simulink model "a_test"  (R2022b)
settings: Solver=VariableStepAuto  StartTime=0.0  StopTime=10.0  RelTol=1e-3
values from neighbouring files (symbols this model uses):
  L = 0.00046    [electric_current_loop.m]    (also in electric_kp_ki.m; pll.m = 10000; sl_ekf.m = c.L_LINE; sl_flux.m = L_avg - 0.5 * L_diff + L_diff * iq_obs * iq_obs / i2_obs)
undefined symbols (not defined in the file or in its folder): D_PI_I, D_PI_KB, D_PI_LOW_LIMIT, D_PI_P, D_PI_UP_LIMIT, Q_PI_I, Q_PI_KB, Q_PI_LOW_LIMIT, Q_PI_P, Q_PI_UP_LIMIT
libraries: slpidlib x6, spsPermanentMagnetSynchronousMachineLib x4, simulink x4, spsDCVoltageSourceLib x2, spsGroundLib x2, spsThreePhaseVIMeasurementLib x2, spsUniversalBridgeLib x2, spspowerguiLib x2
(part 2 of 2)

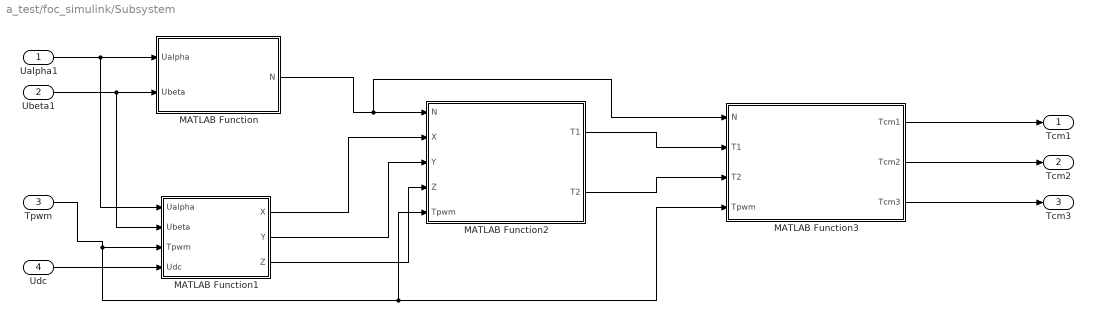
== system a_test/foc_simulink/Subsystem ==
  Ualpha1 : Inport
  Ubeta1 : Inport  Port=2
  Tpwm : Inport  Port=3
  Udc : Inport  Port=4
  MATLAB Function : MATLAB Function  TreatAsAtomicUnit=on
  MATLAB Function1 : MATLAB Function  TreatAsAtomicUnit=on
  MATLAB Function2 : MATLAB Function  TreatAsAtomicUnit=on
  MATLAB Function3 : MATLAB Function  TreatAsAtomicUnit=on
  Tcm1 : Outport
  Tcm2 : Outport  Port=2
  Tcm3 : Outport  Port=3
  wires:
  MATLAB Function3/2(Tcm2) -> Tcm2/1
  Tpwm/1 -> MATLAB Function3/4(Tpwm), MATLAB Function2/5(Tpwm), MATLAB Function1/3(Tpwm)
  MATLAB Function/1(N) -> MATLAB Function3/1(N), MATLAB Function2/1(N)
  Udc/1 -> MATLAB Function1/4(Udc)
  MATLAB Function3/3(Tcm3) -> Tcm3/1
  MATLAB Function2/1(T1) -> MATLAB Function3/2(T1)
  Ualpha1/1 -> MATLAB Function1/1(Ualpha), MATLAB Function/1(Ualpha)
  MATLAB Function2/2(T2) -> MATLAB Function3/3(T2)
  Ubeta1/1 -> MATLAB Function1/2(Ubeta), MATLAB Function/2(Ubeta)
  MATLAB Function3/1(Tcm1) -> Tcm1/1
  MATLAB Function1/1(X) -> MATLAB Function2/2(X)
  MATLAB Function1/3(Z) -> MATLAB Function2/4(Z)
  MATLAB Function1/2(Y) -> MATLAB Function2/3(Y)

== system a_test/foc_simulink/anti_park ==
  Vd : Inport
  Vq : Inport  Port=2
  theta : Inport  Port=3
  MATLAB Function : MATLAB Function  TreatAsAtomicUnit=on
  MATLAB Function1 : MATLAB Function  TreatAsAtomicUnit=on
  Valpha : Outport
  Vbeta : Outport  Port=2
  wires:
  MATLAB Function/1(Valpha) -> Valpha/1
  MATLAB Function1/1(Vbeta) -> Vbeta/1
  Vd/1 -> MATLAB Function/1(Vd), MATLAB Function1/1(Vd)
  Vq/1 -> MATLAB Function/2(Vq), MATLAB Function1/2(Vq)
  theta/1 -> MATLAB Function/3(theta), MATLAB Function1/3(theta)

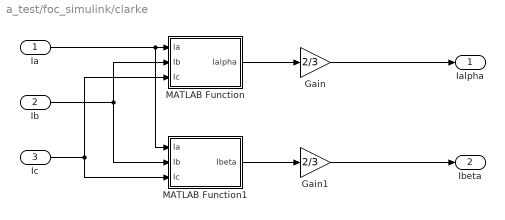
== system a_test/foc_simulink/clarke ==
  Ia : Inport
  Ib : Inport  Port=2
  Ic : Inport  Port=3
  Gain : Gain  Gain=2/3  OutDataTypeStr=single
  Gain1 : Gain  Gain=2/3  OutDataTypeStr=single
  MATLAB Function : MATLAB Function  TreatAsAtomicUnit=on
  MATLAB Function1 : MATLAB Function  TreatAsAtomicUnit=on
  Ialpha : Outport
  Ibeta : Outport  Port=2
  wires:
  Ia/1 -> MATLAB Function1/1(Ia), MATLAB Function/1(Ia)
  MATLAB Function/1(Ialpha) -> Gain/1
  Gain1/1 -> Ibeta/1
  Ib/1 -> MATLAB Function1/2(Ib), MATLAB Function/2(Ib)
  Ic/1 -> MATLAB Function/3(Ic), MATLAB Function1/3(Ic)
  MATLAB Function1/1(Ibeta) -> Gain1/1
  Gain/1 -> Ialpha/1

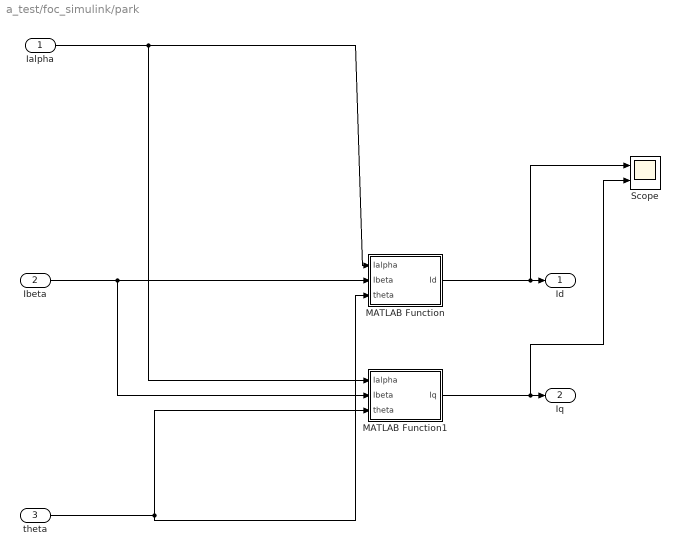
== system a_test/foc_simulink/park ==
  Ialpha : Inport
  Ibeta : Inport  Port=2
  theta : Inport  Port=3
  MATLAB Function : MATLAB Function  TreatAsAtomicUnit=on
  MATLAB Function1 : MATLAB Function  TreatAsAtomicUnit=on
  Scope : Scope  NumInputPorts=2
  Id : Outport
  Iq : Outport  Port=2
  wires:
  theta/1 -> MATLAB Function/3(theta), MATLAB Function1/3(theta)
  Ibeta/1 -> MATLAB Function/2(Ibeta), MATLAB Function1/2(Ibeta)
  MATLAB Function1/1(Iq) -> Scope/2, Iq/1
  MATLAB Function/1(Id) -> Scope/1, Id/1
  Ialpha/1 -> MATLAB Function/1(Ialpha), MATLAB Function1/1(Ialpha)

== system a_test/foc_simulink1/anti_park ==
  Vd : Inport
  Vq : Inport  Port=2
  theta : Inport  Port=3
  antipark_valpha_fun : MATLAB Function  TreatAsAtomicUnit=on
  antipark_vbeta_fun : MATLAB Function  TreatAsAtomicUnit=on
  Valpha : Outport
  Vbeta : Outport  Port=2
  wires:
  antipark_valpha_fun/1(Valpha) -> Valpha/1
  antipark_vbeta_fun/1(Vbeta) -> Vbeta/1
  Vd/1 -> antipark_valpha_fun/1(Vd), antipark_vbeta_fun/1(Vd)
  Vq/1 -> antipark_valpha_fun/2(Vq), antipark_vbeta_fun/2(Vq)
  theta/1 -> antipark_valpha_fun/3(theta), antipark_vbeta_fun/3(theta)

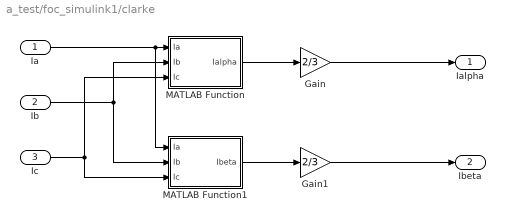
== system a_test/foc_simulink1/clarke ==
  Ia : Inport
  Ib : Inport  Port=2
  Ic : Inport  Port=3
  Gain : Gain  Gain=2/3  OutDataTypeStr=single
  Gain1 : Gain  Gain=2/3  OutDataTypeStr=single
  MATLAB Function : MATLAB Function  TreatAsAtomicUnit=on
  MATLAB Function1 : MATLAB Function  TreatAsAtomicUnit=on
  Ialpha : Outport
  Ibeta : Outport  Port=2
  wires:
  Ia/1 -> MATLAB Function1/1(Ia), MATLAB Function/1(Ia)
  MATLAB Function/1(Ialpha) -> Gain/1
  Gain1/1 -> Ibeta/1
  Ib/1 -> MATLAB Function1/2(Ib), MATLAB Function/2(Ib)
  Ic/1 -> MATLAB Function/3(Ic), MATLAB Function1/3(Ic)
  MATLAB Function1/1(Ibeta) -> Gain1/1
  Gain/1 -> Ialpha/1

== system a_test/foc_simulink1/park ==
  Ialpha : Inport
  Ibeta : Inport  Port=2
  theta : Inport  Port=3
  Scope : Scope  NumInputPorts=2
  park_id_fun : MATLAB Function  TreatAsAtomicUnit=on
  park_iq_fun : MATLAB Function  TreatAsAtomicUnit=on
  Id : Outport
  Iq : Outport  Port=2
  wires:
  theta/1 -> park_id_fun/3(theta), park_iq_fun/3(theta)
  Ibeta/1 -> park_id_fun/2(Ibeta), park_iq_fun/2(Ibeta)
  park_iq_fun/1(Iq) -> Scope/2, Iq/1
  park_id_fun/1(Id) -> Scope/1, Id/1
  Ialpha/1 -> park_id_fun/1(Ialpha), park_iq_fun/1(Ialpha)

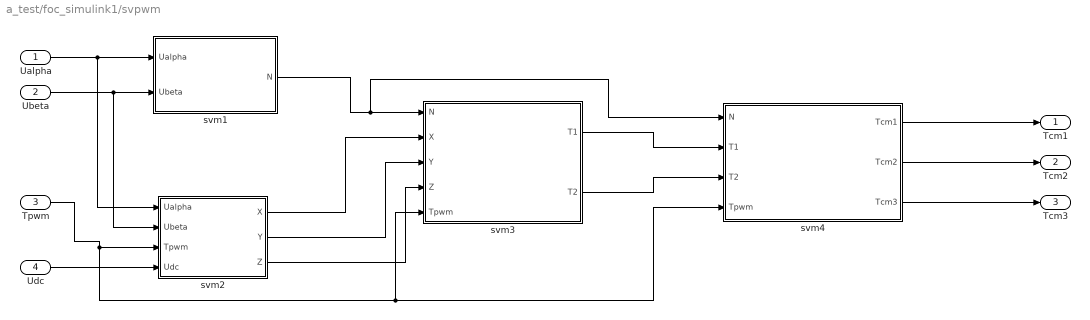
== system a_test/foc_simulink1/svpwm ==
  Ualpha : Inport
  Ubeta : Inport  Port=2
  Tpwm : Inport  Port=3
  Udc : Inport  Port=4
  svm1 : MATLAB Function  TreatAsAtomicUnit=on
  svm2 : MATLAB Function  TreatAsAtomicUnit=on
  svm3 : MATLAB Function  TreatAsAtomicUnit=on
  svm4 : MATLAB Function  TreatAsAtomicUnit=on
  Tcm1 : Outport
  Tcm2 : Outport  Port=2
  Tcm3 : Outport  Port=3
  wires:
  svm4/2(Tcm2) -> Tcm2/1
  Tpwm/1 -> svm4/4(Tpwm), svm3/5(Tpwm), svm2/3(Tpwm)
  svm1/1(N) -> svm4/1(N), svm3/1(N)
  Udc/1 -> svm2/4(Udc)
  svm4/3(Tcm3) -> Tcm3/1
  svm3/1(T1) -> svm4/2(T1)
  Ualpha/1 -> svm2/1(Ualpha), svm1/1(Ualpha)
  svm3/2(T2) -> svm4/3(T2)
  Ubeta/1 -> svm2/2(Ubeta), svm1/2(Ubeta)
  svm4/1(Tcm1) -> Tcm1/1
  svm2/1(X) -> svm3/2(X)
  svm2/3(Z) -> svm3/4(Z)
  svm2/2(Y) -> svm3/3(Y)

== matlab function a_test/foc_simulink/Subsystem/MATLAB Function3 ==
  data: N input; Tcm1 output; T1 input; T2 input; Tpwm input; Tcm2 output; Tcm3 output
function [Tcm1, Tcm2, Tcm3] = fcn(N, T1, T2, Tpwm)

Tcm1 = single(0);
Tcm2 = single(0);
Tcm3 = single(0);


if N == 1
    Tcm1 = (Tpwm + T1 - T2) / 4;
    Tcm2 = (Tpwm - T1 - T2) / 4;
    Tcm3 = (Tpwm + T1 + T2) / 4;
elseif N == 2
    Tcm1 = (Tpwm - T1 - T2) / 4;
    Tcm2 = (Tpwm + T1 + T2) / 4;
    Tcm3 = (Tpwm + T1 - T2) / 4;
elseif N == 3
    Tcm1 = (Tpwm - T1 - T2) / 4;
    Tcm2 = (Tpwm + T1 - T2) / 4;
    Tcm3 = (Tpwm + T1 + T2) / 4;
elseif N == 4
    Tcm1 = (Tpwm + T1 + T2) / 4;
    Tcm2 = (Tpwm + T1 - T2) / 4;
    Tcm3 = (Tpwm - T1 - T2) / 4;
elseif N == 5
    Tcm1 = (Tpwm + T1 + T2) / 4;
    Tcm2 = (Tpwm - T1 - T2) / 4;
    Tcm3 = (Tpwm + T1 - T2) / 4;
elseif N == 6
    Tcm1 = (Tpwm + T1 - T2) / 4;
    Tcm2 = (Tpwm + T1 + T2) / 4;
    Tcm3 = (Tpwm - T1 - T2) / 4;
end

== matlab function a_test/foc_simulink1/anti_park/antipark_valpha_fun ==
  data: Vd input; Valpha output; Vq input; theta input
function Valpha = fcn(Vd, Vq, theta)

Valpha = Vd * cos(theta) - Vq * sin(theta);

== matlab function a_test/foc_simulink1/MATLAB Function2 ==
  data: We input; y output; Iq input
function y = fcn(We, Iq)

% y = -We * Lq * Iq;
y = -We * 1.4e-3 * Iq;

== matlab function a_test/foc_simulink/anti_park/MATLAB Function1 ==
  data: Vd input; Vbeta output; Vq input; theta input
function Vbeta = fcn(Vd, Vq, theta)

Vbeta = Vd * sin(theta) + Vq * cos(theta);

== matlab function a_test/foc_simulink1/MATLAB Function3 ==
  data: We input; y output; Id input
function y = fcn(We, Id)

% y = We * (Flux + Ld * Id);  
y = We * (0.034182 + 1.4e-3 * Id);

== matlab function a_test/foc_simulink1/anti_park/antipark_vbeta_fun ==
  data: Vd input; Vbeta output; Vq input; theta input
function Vbeta = fcn(Vd, Vq, theta)

Vbeta = Vd * sin(theta) + Vq * cos(theta);

== matlab function a_test/foc_simulink1/clarke/MATLAB Function ==
  data: Ia input; Ialpha output; Ib input; Ic input
function Ialpha = fcn(Ia, Ib, Ic)

Ialpha = 3/2 * Ia;

== matlab function a_test/foc_simulink1/clarke/MATLAB Function1 ==
  data: Ia input; Ibeta output; Ib input; Ic input
function Ibeta = fcn( Ia, Ib, Ic)

Ibeta = sqrt(3)/2 * (Ia + 2 * Ib);

== matlab function a_test/foc_simulink1/park/park_id_fun ==
  data: Ialpha input; Id output; Ibeta input; theta input
function Id = fcn(Ialpha, Ibeta, theta)

Id = Ialpha * cos(theta) + Ibeta * sin(theta);

== matlab function a_test/foc_simulink1/park/park_iq_fun ==
  data: Ialpha input; Iq output; Ibeta input; theta input
function Iq = fcn(Ialpha, Ibeta, theta)
Iq = -Ialpha * sin(theta) + Ibeta * cos(theta);

== matlab function a_test/foc_simulink1/svpwm/svm1 ==
  data: Ualpha input; N output; Ubeta input
function N = fcn(Ualpha, Ubeta)

U1 = Ubeta;
U2 = sqrt(3) * Ualpha - Ubeta;
U3 = -sqrt(3) * Ualpha - Ubeta;
A = 0;
B = 0;
C = 0;

if U1 > 0
    A = 1;
else
    A = 0;
end

if U2 > 0
    B = 1;
else
    B = 0;
end

if U3 > 0
    C = 1;
else
    C = 0;
end

N = A + 2 * B + 4 * C;

== matlab function a_test/foc_simulink/clarke/MATLAB Function ==
  data: Ia input; Ialpha output; Ib input; Ic input
function Ialpha = fcn(Ia, Ib, Ic)

Ialpha = 3/2 * Ia;

== matlab function a_test/foc_simulink/clarke/MATLAB Function1 ==
  data: Ia input; Ibeta output; Ib input; Ic input
function Ibeta = fcn( Ia, Ib, Ic)

Ibeta = sqrt(3)/2 * (Ia + 2 * Ib);

== matlab function a_test/foc_simulink/park/MATLAB Function ==
  data: Ialpha input; Id output; Ibeta input; theta input
function Id = fcn(Ialpha, Ibeta, theta)

Id = Ialpha * cos(theta) + Ibeta * sin(theta);

== matlab function a_test/foc_simulink/anti_park/MATLAB Function ==
  data: Vd input; Valpha output; Vq input; theta input
function Valpha = fcn(Vd, Vq, theta)

Valpha = Vd * cos(theta) - Vq * sin(theta);

== matlab function a_test/foc_simulink/park/MATLAB Function1 ==
  data: Ialpha input; Iq output; Ibeta input; theta input
function Iq = fcn(Ialpha, Ibeta, theta)
Iq = -Ialpha * sin(theta) + Ibeta * cos(theta);

== matlab function a_test/foc_simulink1/svpwm/svm2 ==
  data: Ualpha input; Ubeta input; Tpwm input; Udc input; X output; Y output; Z output
function [X, Y, Z] = fcn(Ualpha, Ubeta, Tpwm, Udc)

X = sqrt(3) * Tpwm * Ubeta / Udc;
Y = sqrt(3) * Tpwm / Udc * (sqrt(3) / 2 * Ualpha + 1 / 2 * Ubeta);
Z = sqrt(3) * Tpwm / Udc * (-sqrt(3) / 2 * Ualpha + 1 / 2 * Ubeta);

== matlab function a_test/foc_simulink1/svpwm/svm3 ==
  data: N input; T1 output; X input; Y input; Z input; Tpwm input; T2 output
function [T1, T2] = fcn(N, X, Y, Z, Tpwm)

T1 = single(0);
T2 = single(0);

if N == 1
    T1 = Z;
    T2 = Y;
elseif N == 2
    T1 = Y;
    T2 = -X;
elseif N == 3
    T1 = -Z;
    T2 = X;
elseif N == 4
    T1 = -X;
    T2 = Z;
elseif N == 5
    T1 = X;
    T2 = -Y;
elseif N == 6
    T1 = -Y;
    T2 = -Z;
end

== matlab function a_test/foc_simulink1/svpwm/svm4 ==
  data: N input; Tcm1 output; T1 input; T2 input; Tpwm input; Tcm2 output; Tcm3 output
function [Tcm1, Tcm2, Tcm3] = fcn(N, T1, T2, Tpwm)

Tcm1 = single(0);
Tcm2 = single(0);
Tcm3 = single(0);


if N == 1
    Tcm1 = (Tpwm + T1 - T2) / 4;
    Tcm2 = (Tpwm - T1 - T2) / 4;
    Tcm3 = (Tpwm + T1 + T2) / 4;
elseif N == 2
    Tcm1 = (Tpwm - T1 - T2) / 4;
    Tcm2 = (Tpwm + T1 + T2) / 4;
    Tcm3 = (Tpwm + T1 - T2) / 4;
elseif N == 3
    Tcm1 = (Tpwm - T1 - T2) / 4;
    Tcm2 = (Tpwm + T1 - T2) / 4;
    Tcm3 = (Tpwm + T1 + T2) / 4;
elseif N == 4
    Tcm1 = (Tpwm + T1 + T2) / 4;
    Tcm2 = (Tpwm + T1 - T2) / 4;
    Tcm3 = (Tpwm - T1 - T2) / 4;
elseif N == 5
    Tcm1 = (Tpwm + T1 + T2) / 4;
    Tcm2 = (Tpwm - T1 - T2) / 4;
    Tcm3 = (Tpwm + T1 - T2) / 4;
elseif N == 6
    Tcm1 = (Tpwm + T1 - T2) / 4;
    Tcm2 = (Tpwm + T1 + T2) / 4;
    Tcm3 = (Tpwm - T1 - T2) / 4;
end

== matlab function a_test/Subsystem1/SVPWM ==
  data: Alpha input; A output; B output; C output; Sector output; Beta input; PWMFullDutyCycle input
function [A, B, C, Sector] = fcn(Alpha, Beta, PWMFullDutyCycle)

% 初始化变量
A = single(0);
B = single(0);
C = single(0);                                  
Sector = 0;
ONE_BY_SQRT3 = tand(30);
TWO_BY_SQRT3 = (2.0 * 0.57735026919);

% 扇区判断
if Beta >= 0.0
    if Alpha >= 0.0
        if (ONE_BY_SQRT3 * Beta) > Alpha
                Sector = 2;
        else
            Sector = 1;
        end
    else
        if -ONE_BY_SQRT3 * Beta > Alpha
            Sector = 3;
        else
            Sector = 2;
        end
    end
else
    if Alpha >= 0.0
        if -ONE_BY_SQRT3 * Beta > Alpha
            Sector = 5;
        else
            Sector = 6;
        end

    else
        if ONE_BY_SQRT3 * Beta > Alpha
            Sector = 4;
        else
            Sector = 5;
        end
    end
end


switch Sector
    case 1
        t1 = (Alpha - ONE_BY_SQRT3 * Beta) * PWMFullDutyCycle;
        t2 = (TWO_BY_SQRT3 * Beta) * PWMFullDutyCycle;

        A = (PWMFullDutyCycle + t1 + t2) / 2;
        B = A - t1;
        C = B - t2;
    case 2
		t2 = (Alpha + ONE_BY_SQRT3 * Beta) * PWMFullDutyCycle;
		t3 = (-Alpha + ONE_BY_SQRT3 * Beta) * PWMFullDutyCycle;

		B = (PWMFullDutyCycle + t2 + t3) / 2;
		A = B - t3;
		C = A - t2;
        
    case 3
       t3 = (TWO_BY_SQRT3 * Beta) * PWMFullDutyCycle;
		t4 = (-Alpha - ONE_BY_SQRT3 * Beta) * PWMFullDutyCycle;

		B = (PWMFullDutyCycle + t3 + t4) / 2;
		C = B - t3;
		A = C - t4;

    case 4
		t4 = (-Alpha + ONE_BY_SQRT3 * Beta) * PWMFullDutyCycle;
		t5 = (-TWO_BY_SQRT3 * Beta) * PWMFullDutyCycle;

		C = (PWMFullDutyCycle + t4 + t5) / 2;
		B = C - t5;
		A = B - t4;
    case 5
        t5 = (-Alpha - ONE_BY_SQRT3 * Beta) * PWMFullDutyCycle;
		t6 = (Alpha - ONE_BY_SQRT3 * Beta) * PWMFullDutyCycle;

		C = (PWMFullDutyCycle + t5 + t6) / 2;
		A = C - t5;
		B = A - t6;

    case 6
		t6 = (-TWO_BY_SQRT3 * Beta) * PWMFullDutyCycle;
		t1 = (Alpha + ONE_BY_SQRT3 * Beta) * PWMFullDutyCycle;

		A = (PWMFullDutyCycle + t6 + t1) / 2;
		C = A - t1;
		B = C - t6;
end

== matlab function a_test/foc_simulink/MATLAB Function ==
  data: we input; y output; Id input
function y = fcn(we, Id)

% 磁链和电感 %

y = we * (0.034182 + 1.4e-3 * Id);

== matlab function a_test/foc_simulink/MATLAB Function1 ==
  data: we input; y output; Iq input
function y = fcn(we, Iq)

y = -we * Iq * 0.034182;

== matlab function a_test/Subsystem2/SVPWM ==
  data: Alpha input; A output; B output; C output; Sector output; Beta input; PWMFullDutyCycle input
function [A, B, C, Sector] = fcn(Alpha, Beta, PWMFullDutyCycle)

% 初始化变量
A = single(0);
B = single(0);
C = single(0);                                  
Sector = 0;
ONE_BY_SQRT3 = tand(30);
TWO_BY_SQRT3 = (2.0 * 0.57735026919);

% 扇区判断
if Beta >= 0.0
    if Alpha >= 0.0
        if (ONE_BY_SQRT3 * Beta) > Alpha
                Sector = 2;
        else
            Sector = 1;
        end
    else
        if -ONE_BY_SQRT3 * Beta > Alpha
            Sector = 3;
        else
            Sector = 2;
        end
    end
else
    if Alpha >= 0.0
        if -ONE_BY_SQRT3 * Beta > Alpha
            Sector = 5;
        else
            Sector = 6;
        end

    else
        if ONE_BY_SQRT3 * Beta > Alpha
            Sector = 4;
        else
            Sector = 5;
        end
    end
end


switch Sector
    case 1
        t1 = (Alpha - ONE_BY_SQRT3 * Beta) * PWMFullDutyCycle;
        t2 = (TWO_BY_SQRT3 * Beta) * PWMFullDutyCycle;

        A = (PWMFullDutyCycle + t1 + t2) / 2;
        B = A - t1;
        C = B - t2;
    case 2
		t2 = (Alpha + ONE_BY_SQRT3 * Beta) * PWMFullDutyCycle;
		t3 = (-Alpha + ONE_BY_SQRT3 * Beta) * PWMFullDutyCycle;

		B = (PWMFullDutyCycle + t2 + t3) / 2;
		A = B - t3;
		C = A - t2;
        
    case 3
       t3 = (TWO_BY_SQRT3 * Beta) * PWMFullDutyCycle;
		t4 = (-Alpha - ONE_BY_SQRT3 * Beta) * PWMFullDutyCycle;

		B = (PWMFullDutyCycle + t3 + t4) / 2;
		C = B - t3;
		A = C - t4;

    case 4
		t4 = (-Alpha + ONE_BY_SQRT3 * Beta) * PWMFullDutyCycle;
		t5 = (-TWO_BY_SQRT3 * Beta) * PWMFullDutyCycle;

		C = (PWMFullDutyCycle + t4 + t5) / 2;
		B = C - t5;
		A = B - t4;
    case 5
        t5 = (-Alpha - ONE_BY_SQRT3 * Beta) * PWMFullDutyCycle;
		t6 = (Alpha - ONE_BY_SQRT3 * Beta) * PWMFullDutyCycle;

		C = (PWMFullDutyCycle + t5 + t6) / 2;
		A = C - t5;
		B = A - t6;

    case 6
		t6 = (-TWO_BY_SQRT3 * Beta) * PWMFullDutyCycle;
		t1 = (Alpha + ONE_BY_SQRT3 * Beta) * PWMFullDutyCycle;

		A = (PWMFullDutyCycle + t6 + t1) / 2;
		C = A - t1;
		B = C - t6;
end

== matlab function a_test/foc_simulink/Subsystem/MATLAB Function ==
  data: Ualpha input; N output; Ubeta input
function N = fcn(Ualpha, Ubeta)

U1 = Ubeta;
U2 = sqrt(3) * Ualpha - Ubeta;
U3 = -sqrt(3) * Ualpha - Ubeta;
A = 0;
B = 0;
C = 0;

if U1 > 0
    A = 1;
else
    A = 0;
end

if U2 > 0
    B = 1;
else
    B = 0;
end

if U3 > 0
    C = 1;
else
    C = 0;
end

N = A + 2 * B + 4 * C;

== matlab function a_test/foc_simulink/Subsystem/MATLAB Function1 ==
  data: Ualpha input; Ubeta input; Tpwm input; Udc input; X output; Y output; Z output
function [X, Y, Z] = fcn(Ualpha, Ubeta, Tpwm, Udc)

X = sqrt(3) * Tpwm * Ubeta / Udc;
Y = sqrt(3) * Tpwm / Udc * (sqrt(3) / 2 * Ualpha + 1 / 2 * Ubeta);
Z = sqrt(3) * Tpwm / Udc * (-sqrt(3) / 2 * Ualpha + 1 / 2 * Ubeta);

== matlab function a_test/foc_simulink/Subsystem/MATLAB Function2 ==
  data: N input; T1 output; X input; Y input; Z input; Tpwm input; T2 output
function [T1, T2] = fcn(N, X, Y, Z, Tpwm)

T1 = single(0);
T2 = single(0);

if N == 1
    T1 = Z;
    T2 = Y;
elseif N == 2
    T1 = Y;
    T2 = -X;
elseif N == 3
    T1 = -Z;
    T2 = X;
elseif N == 4
    T1 = -X;
    T2 = Z;
elseif N == 5
    T1 = X;
    T2 = -Y;
elseif N == 6
    T1 = -Y;
    T2 = -Z;
end
